simulink model "MyHistogramEqualization"  (R2024b)
settings: Solver=VariableStepAuto  StartTime=0.0  StopTime=10.0  RelTol=1e-3
undefined symbols (not defined in the file): Rec, SDTV
libraries: visionconversions x2, visionanalysis x1, visionsources x1
settings Model: Creator=snmz4  LastModifiedBy=snmz4

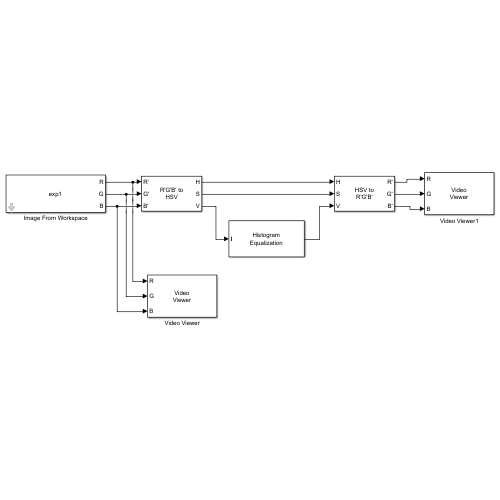
[thumbnail: Simulink's stored preview of the top-level diagram]
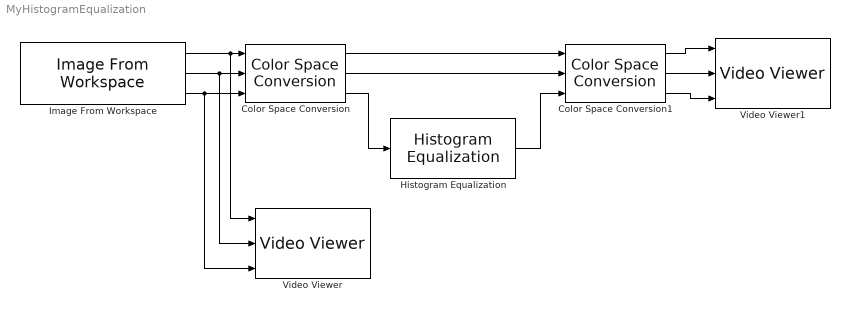
== system MyHistogramEqualization ==
  Color Space Conversion : visionconversions/Color Space  Conversion  conversion=Obsolete  conversionActive=R'G'B' to HSV  wp_str=D65  rec=Rec. 601 (SDTV)  sys=1125/60/2:1  imagePorts=Separate color signals
  Color Space Conversion1 : visionconversions/Color Space  Conversion  conversion=Obsolete  conversionActive=HSV to R'G'B'  wp_str=D65  rec=Rec. 601 (SDTV)  sys=1125/60/2:1  imagePorts=Separate color signals
  Histogram Equalization : visionanalysis/Histogram Equalization  specify=Uniform  numbins=64  src=Specify via dialog  hist=ones(1,64)
  Image From Workspace : visionsources/Image From Workspace  Tag=vipblks_nd  ImageValue=exp1  Ts=inf  imagePorts=Separate color signals  OutPortLabels=R|G|B  ImageDataType=double  Signed=on  WordLength=16  sdImageDataType=sfix(16)  FractionLengthMode=User-defined  FractionLength=15
  Video Viewer : VideoViewer  imagePorts=separate color signals  FigPos=[530.6 578 417.6 304]
  Video Viewer1 : VideoViewer  imagePorts=separate color signals  FigPos=[974.6 580.4 417.6 304]
  wires:
  Image From Workspace/1 -> Video Viewer/1, Color Space Conversion/1
  Image From Workspace/2 -> Color Space Conversion/2, Video Viewer/2
  Image From Workspace/3 -> Color Space Conversion/3, Video Viewer/3
  Color Space Conversion/3 -> Histogram Equalization/1
  Histogram Equalization/1 -> Color Space Conversion1/3
  Color Space Conversion/1 -> Color Space Conversion1/1
  Color Space Conversion/2 -> Color Space Conversion1/2
  Color Space Conversion1/1 -> Video Viewer1/1
  Color Space Conversion1/2 -> Video Viewer1/2
  Color Space Conversion1/3 -> Video Viewer1/3
